simulink model "LLC"  (R2024a)
settings: Solver=VariableStepAuto  StartTime=0.0  StopTime=0.05  RelTol=1e-3
libraries: spsSeriesRLCBranchLib x5, spsVoltageMeasurementLib x5, spsDiodeLib x4, spsMosfetLib x4, spsCurrentMeasurementLib x3, spsDCVoltageSourceLib x1, spsLinearTransformerLib x1, spspowerguiLib x1
settings Model: Creator=DIPAK PRODHANI  LastModifiedBy=DIPAK PRODHANI

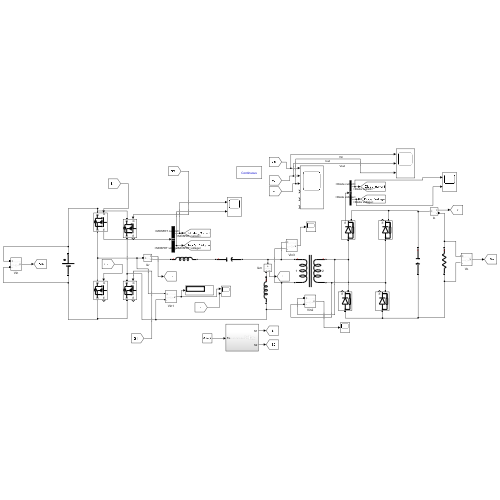
[thumbnail: Simulink's stored preview of the top-level diagram]
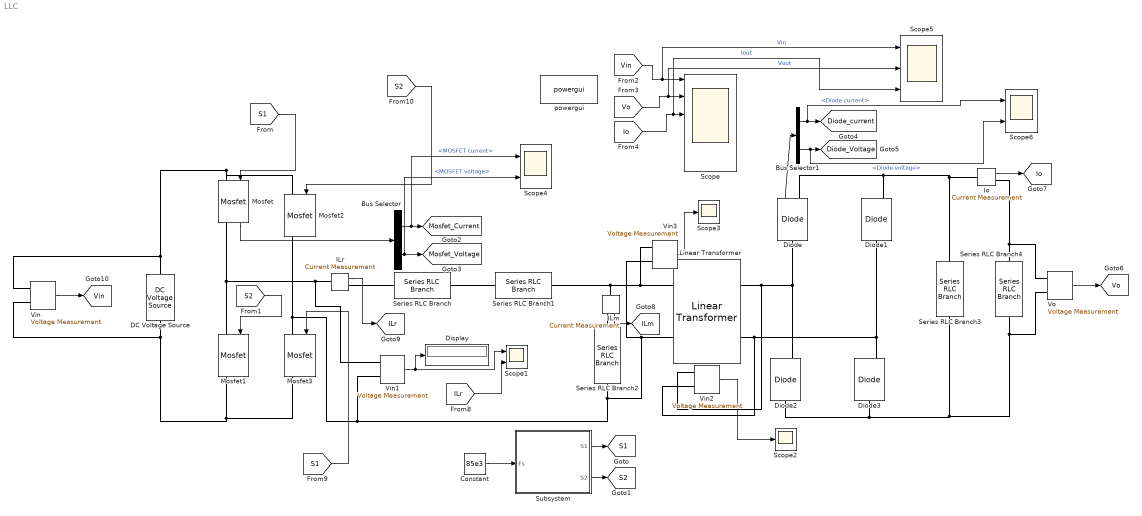
== system LLC ==
  Bus Selector : BusSelector  OutputSignals=MOSFET current,MOSFET voltage
  Bus Selector1 : BusSelector  OutputSignals=Diode current,Diode voltage
  Constant : Constant  Value=85e3
  DC Voltage Source : spsDCVoltageSourceLib/DC Voltage Source  Amplitude=400  Measurements=None
  Diode{,1..3} (4 alike) : spsDiodeLib/Diode  Ron=0.001  Lon=0  Vf=0.8  IC=0  UseSnubber=0  Rs=500  Cs=250e-9  Measurements=on
  Display : Display
  ILm : spsCurrentMeasurementLib/Current Measurement  PhasorSimulation=off  OutputType=Complex  PSBequivalent=0
  ILr : spsCurrentMeasurementLib/Current Measurement  PhasorSimulation=off  OutputType=Complex  PSBequivalent=0
  Io : spsCurrentMeasurementLib/Current Measurement  PhasorSimulation=off  OutputType=Complex  PSBequivalent=0
  Linear Transformer : spsLinearTransformerLib/Linear Transformer  UNITS=SI  NominalPower=[ 700 100e3 ]  winding1=[400 0 0]  winding2=[400 0 0]  ThreeWindings=off  winding3=[3.15e+05 0.7938 0.084225]  RmLm=[100 0]  Measurements=None  DataType=on
  Mosfet{,1..3} (4 alike) : spsMosfetLib/Mosfet  Ron=0.1  Lon=0  Rd=0.01  Vfd=0  IC=0  Rs=1e5  Cs=inf  Measurements=on
  Scope : Scope  NumInputPorts=6
  Scope1 : Scope  NumInputPorts=2
  Scope2 : Scope
  Scope3 : Scope
  Scope4 : Scope  NumInputPorts=2
  Scope5 : Scope  NumInputPorts=3
  Scope6 : Scope  NumInputPorts=2
  Series RLC Branch : spsSeriesRLCBranchLib/Series RLC Branch  LConnTagsString=__new0  RConnTagsString=__new0  BranchType=L  Resistance=1  Inductance=26.59e-6  SetiL0=off  InitialCurrent=0  Capacitance=1e-6  Setx0=off  InitialVoltage=0  Measurements=None
  Series RLC Branch1 : spsSeriesRLCBranchLib/Series RLC Branch  LConnTagsString=__new0  RConnTagsString=__new0  BranchType=C  Resistance=1  Inductance=1e-3  SetiL0=off  InitialCurrent=0  Capacitance=131.76e-9  Setx0=off  InitialVoltage=0  Measurements=None
  Series RLC Branch2 : spsSeriesRLCBranchLib/Series RLC Branch  LConnTagsString=__new0  RConnTagsString=__new0  BranchType=L  Resistance=1  Inductance=93.06e-6  SetiL0=off  InitialCurrent=0  Capacitance=1e-6  Setx0=off  InitialVoltage=0  Measurements=None
  Series RLC Branch3 : spsSeriesRLCBranchLib/Series RLC Branch  LConnTagsString=__new0  RConnTagsString=__new0  BranchType=C  Resistance=1  Inductance=1e-3  SetiL0=off  InitialCurrent=0  Capacitance=100e-6  Setx0=off  InitialVoltage=0  Measurements=None
  Series RLC Branch4 : spsSeriesRLCBranchLib/Series RLC Branch  LConnTagsString=__new0  RConnTagsString=__new0  BranchType=R  Resistance=48.48  Inductance=1e-3  SetiL0=off  InitialCurrent=0  Capacitance=1e-6  Setx0=off  InitialVoltage=0  Measurements=None
  Subsystem : Subsystem
  Vin{,1..3} (4 alike) : spsVoltageMeasurementLib/Voltage Measurement  PhasorSimulation=off  OutputType=Complex  PSBequivalent=0
  Vo : spsVoltageMeasurementLib/Voltage Measurement  PhasorSimulation=off  OutputType=Complex  PSBequivalent=0
  powergui : spspowerguiLib/powergui  Priority=1  SimulationMode=Continuous  SampleTime=50e-6  frequency=60  Iterations=50  frequencyindice=0  Pbase=100e6  ErrMax=1e-4  UnitsV=kV  UnitsW=MW  buscounter=0  FunctionMessages=off  echomessages=off  EnableUseOfTLC=off  CurrentSourceSwitches=off  DisableSnubberDevices=off  DisableRonSwitches=off  DisableVfSwitches=off  DisplayEquations=off  AutomaticDiscreteSolvers=off  SolverType=Tustin/Backward Euler (TBE)  Interpol=off  ExternalGateDelay=off  methode=off  Ts=100  x0status=blocks  SPID=on  SwTol=0  HookPort=off  NonlinearTolerance=1e-4  nMaxIteration=100  ContinueOnMaxIteration=off  RestoreLinks=warning  ResistiveCurrentMeasurement=off  Frange=[0:2:500]  Ylog=off  Xlog=on  ShowGrid=off  save=off  variable=ZData  structure=0  ZoomFFT=off  StartTime=0.0  cycles=1  DisplayStyle=1  fundamental=60  FreqAxis=off  MaxFrequency=1000  frequencyindicesteady=1  RmsSteady=1  display=off
  tag scope: Diode_Voltage=global, Diode_current=global, ILm=global, ILr=global, Io=global, Mosfet_Current=global, Mosfet_Voltage=global, S1=global, S2=global, Vin=global, Vo=global
  wires:
  Subsystem/1(S1) -> [S1]
  Subsystem/2(S2) -> [S2]
  [S1] -> Mosfet/1
  [S2] -> Mosfet1/1
  Mosfet/1 -> Bus Selector/1
  Diode/1 -> Bus Selector1/1
  Bus Selector1/2 -> Scope6/2, [Diode_Voltage]  "<Diode voltage>"
  Bus Selector/2 -> Scope4/2, [Mosfet_Voltage]  "<MOSFET voltage>"
  Bus Selector/1 -> Scope4/1, [Mosfet_Current]  "<MOSFET current>"
  Bus Selector1/1 -> Scope6/1, [Diode_current]  "<Diode current>"
  Vo/1 -> [Vo]
  Io/1 -> [Io]
  ILm/1 -> [ILm]
  ILr/1 -> [ILr]
  Vin/1 -> [Vin]
  [Vin] -> Scope5/1, Scope/1  "Vin"
  [Vo] -> Scope5/2, Scope/2  "Vout"
  [Io] -> Scope5/3, Scope/3  "Iout"
  Constant/1 -> Subsystem/1(Fs)
  Vin1/1 -> Scope1/1, Display/1
  Vin2/1 -> Scope2/1
  Vin3/1 -> Scope3/1
  [ILr] -> Scope1/2
  [S1] -> Mosfet3/1
  [S2] -> Mosfet2/1
  connections:
  Series RLC Branch1/LConn1 -- Series RLC Branch/RConn1
  Linear Transformer/LConn1 -- Vin3/LConn1 -- ILm/LConn1 -- Series RLC Branch1/RConn1
  ILr/LConn1 -- Vin1/LConn1 -- Mosfet1/LConn1 -- Mosfet/RConn1
  DC Voltage Source/RConn1 -- Mosfet2/LConn1 -- Mosfet/LConn1 -- Vin/LConn1
  Diode2/LConn1 -- Series RLC Branch4/RConn1 -- Vo/LConn2 -- Series RLC Branch3/RConn1 -- Diode3/LConn1
  Diode2/RConn1 -- Vin2/LConn1 -- Linear Transformer/RConn1 -- Diode/LConn1
  Diode3/RConn1 -- Vin2/LConn2 -- Linear Transformer/RConn2 -- Diode1/LConn1
  Diode1/RConn1 -- Io/LConn1 -- Series RLC Branch3/LConn1 -- Diode/RConn1
  Io/RConn1 -- Series RLC Branch4/LConn1 -- Vo/LConn1
  ILr/RConn1 -- Series RLC Branch/LConn1
  ILm/RConn1 -- Series RLC Branch2/LConn1
  Mosfet2/RConn1 -- Linear Transformer/LConn2 -- Vin3/LConn2 -- Series RLC Branch2/RConn1 -- Vin1/LConn2 -- Mosfet3/LConn1
  Vin/LConn2 -- Mosfet3/RConn1 -- Mosfet1/RConn1 -- DC Voltage Source/LConn1

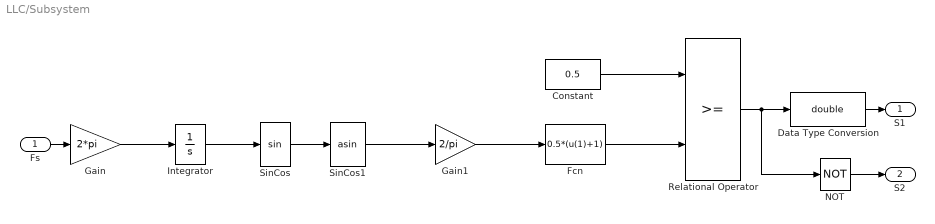
== system LLC/Subsystem ==
  Fs : Inport
  Constant : Constant  Value=0.5
  Data Type Conversion : DataTypeConversion  OutDataTypeStr=double  SaturateOnIntegerOverflow=off  RndMeth=Floor
  Fcn : Fcn  Expr=0.5*(u(1)+1)
  Gain : Gain  Gain=2*pi
  Gain1 : Gain  Gain=2/pi
  Integrator : Integrator
  NOT : Logic  Operator=NOT  IconShape=distinctive  AllPortsSameDT=off  OutDataTypeStr=boolean
  Relational Operator : RelationalOperator  OutDataTypeStr=boolean  RndMeth=Simplest  InputSameDT=off
  SinCos : Trigonometry
  SinCos1 : Trigonometry  Operator=asin
  S1 : Outport
  S2 : Outport  Port=2
  wires:
  SinCos1/1 -> Gain1/1
  Relational Operator/1 -> Data Type Conversion/1, NOT/1
  Gain1/1 -> Fcn/1
  Constant/1 -> Relational Operator/1
  Gain/1 -> Integrator/1
  Data Type Conversion/1 -> S1/1
  Fs/1 -> Gain/1
  Integrator/1 -> SinCos/1
  SinCos/1 -> SinCos1/1
  Fcn/1 -> Relational Operator/2
  NOT/1 -> S2/1
